simulink model "simulink0_full_stateback_control"  (R2026b)
settings: Solver=VariableStepAuto  StopTime=40.0
values from neighbouring files (symbols this model uses):
  K = place(A, B, P)    [full_stateback_control.m]
  kr = 1/dcgain(Sys_cl)    [full_stateback_control.m]
undefined symbols (not defined in the file or in its folder): A, B, C
settings Model: Creator=leelou  LastModifiedBy=leelou

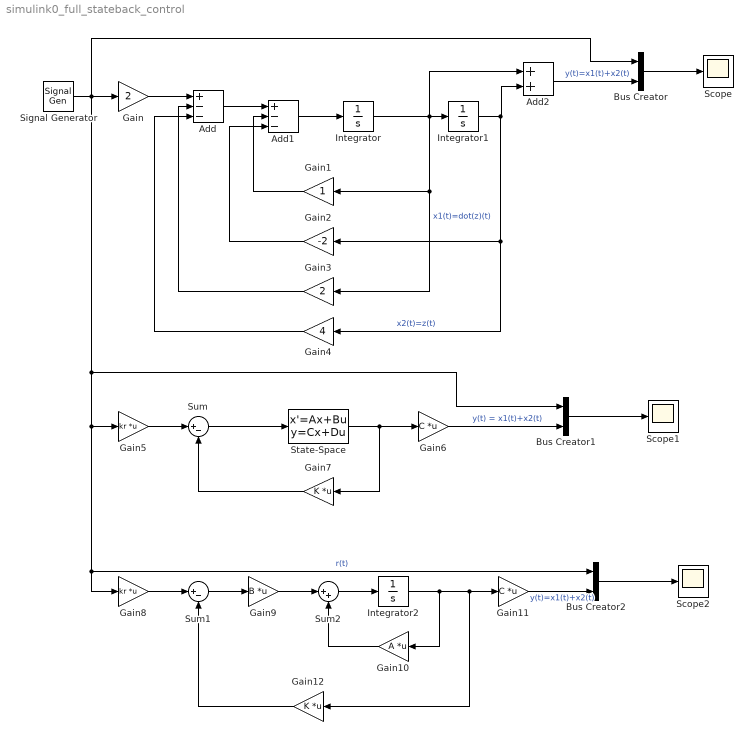
== system simulink0_full_stateback_control ==
  Add : Sum  Inputs=+--
  Add1 : Sum  Inputs=+--
  Add2 : Sum
  Bus Creator : BusCreator  Inputs=2
  Bus Creator1 : BusCreator  Inputs=2
  Bus Creator2 : BusCreator  Inputs=2
  Gain : Gain  Gain=2
  Gain1 : Gain
  Gain10 : Gain  Gain=A  Multiplication=Matrix(K*u)
  Gain11 : Gain  Gain=C  Multiplication=Matrix(K*u)
  Gain12 : Gain  Gain=K  Multiplication=Matrix(K*u)
  Gain2 : Gain  Gain=-2
  Gain3 : Gain  Gain=2
  Gain4 : Gain  Gain=4
  Gain5 : Gain  Gain=kr  Multiplication=Matrix(K*u)
  Gain6 : Gain  Gain=C  Multiplication=Matrix(K*u)
  Gain7 : Gain  Gain=K  Multiplication=Matrix(K*u)
  Gain8 : Gain  Gain=kr  Multiplication=Matrix(K*u)
  Gain9 : Gain  Gain=B  Multiplication=Matrix(K*u)
  Integrator : Integrator
  Integrator1 : Integrator
  Integrator2 : Integrator
  Scope : Scope
      settings: ActiveDisplayYMinimum=-1.25  ActiveDisplayYMaximum=1.25
  Scope1 : Scope
      settings: ActiveDisplayYMinimum=-1.25  ActiveDisplayYMaximum=1.25
  Scope2 : Scope
      settings: ActiveDisplayYMinimum=-1.25  ActiveDisplayYMaximum=1.25  DataLoggingVariableName=ScopeData2
  Signal Generator : SignalGenerator  WaveForm=square  Frequency=1/20
  State-Space : StateSpace  A=A  B=B  C=eye(2)  D=[0;0]  InitialCondition=0
  Sum : Sum  Inputs=|+-
  Sum1 : Sum  Inputs=|+-
  Sum2 : Sum  Inputs=|++
  wires:
  Signal Generator/1 -> Bus Creator1/1, Gain8/1, Bus Creator2/1, Gain5/1, Bus Creator/1, Gain/1  "r(t)"
  Gain/1 -> Add/1
  Add/1 -> Add1/1
  Add1/1 -> Integrator/1
  Gain1/1 -> Add1/2
  Integrator/1 -> Gain3/1, Gain1/1, Add2/1, Integrator1/1  "x1(t)=dot(z)(t)"
  Integrator1/1 -> Gain4/1, Gain2/1, Add2/2  "x2(t)=z(t)"
  Gain2/1 -> Add1/3
  Add2/1 -> Bus Creator/2  "y(t)=x1(t)+x2(t)"
  Bus Creator/1 -> Scope/1
  Gain3/1 -> Add/2
  Gain4/1 -> Add/3
  Gain5/1 -> Sum/1
  Sum/1 -> State-Space/1
  State-Space/1 -> Gain7/1, Gain6/1
  Gain6/1 -> Bus Creator1/2  "y(t) = x1(t)+x2(t)"
  Bus Creator1/1 -> Scope1/1
  Gain7/1 -> Sum/2
  Gain8/1 -> Sum1/1
  Sum1/1 -> Gain9/1
  Gain9/1 -> Sum2/1
  Sum2/1 -> Integrator2/1
  Gain10/1 -> Sum2/2
  Integrator2/1 -> Gain10/1, Gain12/1, Gain11/1
  Gain11/1 -> Bus Creator2/2  "y(t)=x1(t)+x2(t)"
  Bus Creator2/1 -> Scope2/1
  Gain12/1 -> Sum1/2
